simulink model "can2_mcu_imu_pack"  (R2026b)
settings: Solver=VariableStepAuto
undefined symbols (not defined in the file or in its folder): P
libraries: svdutilitieslib x1
settings Model: Creator=aomar  LastModifiedBy=aomar

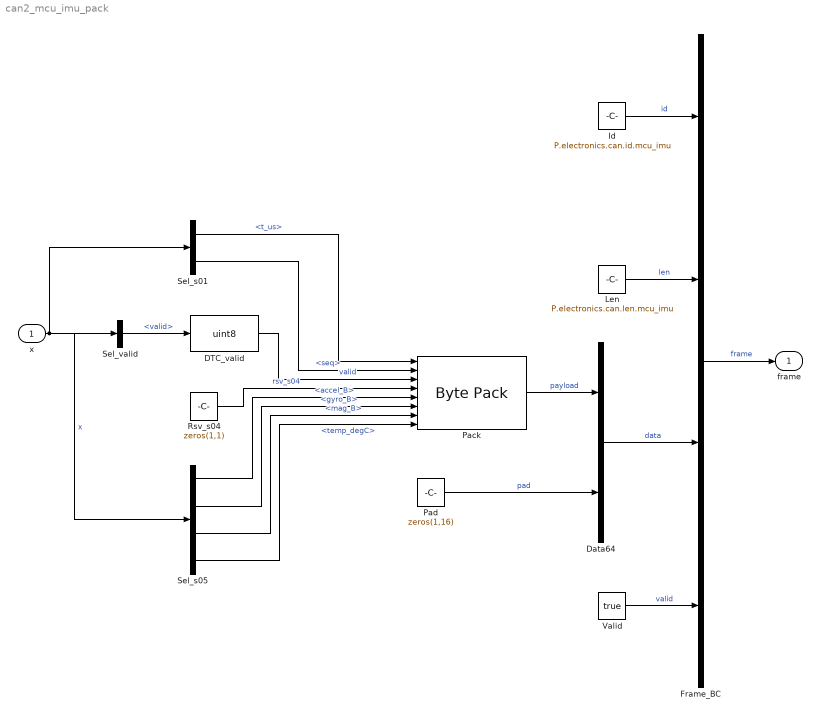
== system can2_mcu_imu_pack ==
  x : Inport  OutDataTypeStr=Bus: Bus_ImuMeas
  DTC_valid : DataTypeConversion  OutDataTypeStr=uint8  RndMeth=Round
  Data64 : Concatenate
  Frame_BC : BusCreator  Inputs=4  OutDataTypeStr=Bus: Bus_CanFrame64  NonVirtualBus=on
      settings: InheritFromInputs=off
  Id : Constant  Value=P.electronics.can.id.mcu_imu  OutDataTypeStr=uint32  SampleTime=-1
  Len : Constant  Value=P.electronics.can.len.mcu_imu  OutDataTypeStr=uint8  SampleTime=-1
  Pack : svdutilitieslib/Byte Pack  maskPackedDataType=uint8  datatypes={'uint32','uint16','uint8','uint8','single','single','single','single'}  byteAlign=1  blockPlatform=arduinoert
      settings: LibrarySourceBlock=mcblib/Signal Management/Byte Pack
  Pad : Constant  Value=zeros(1,16)  OutDataTypeStr=uint8  SampleTime=-1
  Rsv_s04 : Constant  Value=zeros(1,1)  OutDataTypeStr=uint8  SampleTime=-1
  Sel_s01 : BusSelector  OutputSignals=t_us,seq
  Sel_s05 : BusSelector  OutputSignals=accel_B,gyro_B,mag_B,temp_degC
  Sel_valid : BusSelector  OutputSignals=valid
  Valid : Constant  Value=true  OutDataTypeStr=boolean  SampleTime=-1
  frame : Outport  OutDataTypeStr=Bus: Bus_CanFrame64
  wires:
  x/1 -> Sel_s05/1, Sel_s01/1, Sel_valid/1  "x"
  Sel_valid/1 -> DTC_valid/1  "<valid>"
  Sel_s01/1 -> Pack/1  "<t_us>"
  Sel_s01/2 -> Pack/2  "<seq>"
  Sel_s05/1 -> Pack/5  "<accel_B>"
  Sel_s05/2 -> Pack/6  "<gyro_B>"
  Sel_s05/3 -> Pack/7  "<mag_B>"
  Sel_s05/4 -> Pack/8  "<temp_degC>"
  Rsv_s04/1 -> Pack/4  "rsv_s04"
  DTC_valid/1 -> Pack/3  "valid"
  Pad/1 -> Data64/2  "pad"
  Pack/1 -> Data64/1  "payload"
  Data64/1 -> Frame_BC/3  "data"
  Id/1 -> Frame_BC/1  "id"
  Len/1 -> Frame_BC/2  "len"
  Valid/1 -> Frame_BC/4  "valid"
  Frame_BC/1 -> frame/1  "frame"
